simulink model "Harmonic_Restrain_Relay"  (R2024a)
settings: Solver=VariableStepAuto  StartTime=0.0  StopTime=1  EnableMultiTasking=on
libraries: spsFourierLib x4, spsThreePhaseVIMeasurementLib x2, spsThreePhaseBreakerLib x2, spsThreePhaseFaultLib x2, spsCurrentMeasurementLib x1, spsGroundLib x1, spsThreePhaseSeriesRLCBranchLib x1, spsThreePhaseTransformerTwoWindingsLib x1, spsThreePhaseSourceLib x1, spspowerguiLib x1
settings Model: Creator=hp  LastModifiedBy=hp
settings SolverCC: MaxZcPerStep=1
settings DataIOCC: LimitDataPoints=on  MaxDataPoints=10000
settings OptimizationCC: ReuseModelBlockBuffer=off  LifeSpan=inf
settings DebuggingCC: UnconnectedInputMsg=warning  UnconnectedOutputMsg=warning  UnconnectedLineMsg=warning  AllowSymbolicDim=off  SFUnexpectedBacktrackingDiag=warning  SFNoUnconditionalDefaultTransitionDiag=warning  SFExecutionAtInitializationDiag=none  ArithmeticOperatorsInVariantConditions=warning
settings ModelReferenceCC: EnableRefExpFcnMdlSchedulingChecks=on
settings SFSimCC: SimUseLocalCustomCode=off  CustomCodeUndefinedFunction=UseInterfaceOnly
settings RTWCC: RTWUseLocalCustomCode=off  GPUComputeCapability=3.5  DLArmComputeVersion=19.05
settings CodeAppCC: StateflowObjectComments=on
settings GRTTargetCC: TargetLangStandard=C89/C90 (ANSI)
settings ConfigComp: CovMetricSettings=dw  CovSaveCumulativeToWorkspaceVar=on  CovSaveSingleToWorkspaceVar=on  CovExternalEMLEnable=off  CovSFcnEnable=off
settings SimscapeCC: SimscapeLogType=all  SimscapeLogDataHistory=10000

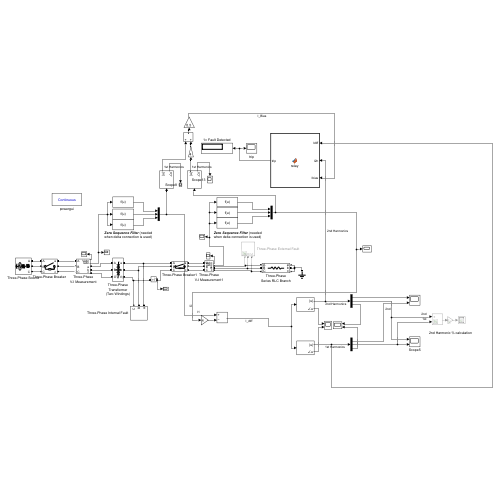
[thumbnail: Simulink's stored preview of the top-level diagram]
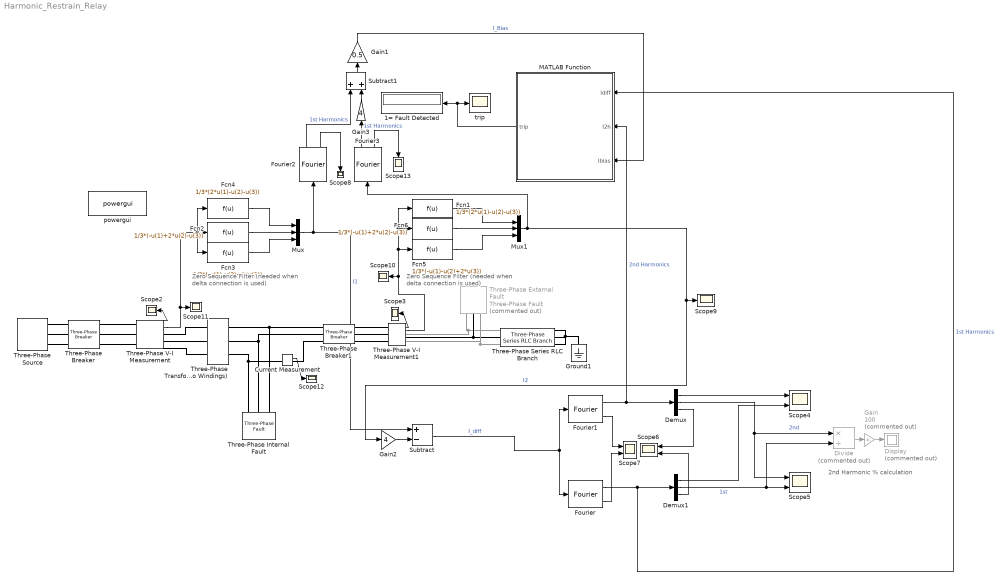
== system Harmonic_Restrain_Relay ==
  note: 2nd Harmonic % calculation
  note: Zero Sequence Filter (needed when delta connection is used)
  note: Zero Sequence Filter (needed when delta connection is used)
  1= Fault Detected : Display
  Current Measurement : spsCurrentMeasurementLib/Current Measurement  PhasorSimulation=off  OutputType=Complex  PSBequivalent=0
  Demux : Demux  Outputs=3
  Demux1 : Demux  Outputs=3
  Display : Display  Commented=on
  Divide : Product  Commented=on  Inputs=*/
  Fcn1 : Fcn  Expr=1/3*(2*u(1)-u(2)-u(3))
  Fcn2 : Fcn  Expr=1/3*(-u(1)+2*u(2)-u(3))
  Fcn3 : Fcn  Expr=1/3*(-u(1)-u(2)+2*u(3))
  Fcn4 : Fcn  Expr=1/3*(2*u(1)-u(2)-u(3))
  Fcn5 : Fcn  Expr=1/3*(-u(1)-u(2)+2*u(3))
  Fcn6 : Fcn  Expr=1/3*(-u(1)+2*u(2)-u(3))
  Fourier : spsFourierLib/Fourier  Freq=60  n=1  InInit=[0, 0]  Ts=0
  Fourier1 : spsFourierLib/Fourier  Freq=60  n=2  InInit=[0, 0]  Ts=0
  Fourier2 : spsFourierLib/Fourier  Freq=60  n=1  InInit=[0, 0]  Ts=0
  Fourier3 : spsFourierLib/Fourier  Freq=60  n=1  InInit=[0, 0]  Ts=0
  Gain : Gain  Commented=on  Gain=100
  Gain1 : Gain  Gain=0.5
  Gain2 : Gain  Gain=4
  Gain3 : Gain  Gain=4
  Ground1 : spsGroundLib/Ground  LConnTagsString=a
  MATLAB Function : MATLAB Function  TreatAsAtomicUnit=on
  Mux : Mux  Inputs=3
  Mux1 : Mux  Inputs=3
  Scope{2..3,8..13} (8 alike) : Scope
  Scope{4..7} (4 alike) : Scope  NumInputPorts=2
  Subtract : Sum  Inputs=+-
  Subtract1 : Sum
  Three-Phase Series RLC Branch : spsThreePhaseSeriesRLCBranchLib/Three-Phase Series RLC Branch  LConnTagsString=A|B|C  RConnTagsString=A|B|C  BranchType=R  Resistance=150  Inductance=0  Capacitance=0  Measurements=None
  Three-Phase Transformer (Two Windings) : spsThreePhaseTransformerTwoWindingsLib/Three-Phase Transformer (Two Windings)  Winding1Connection=Yg  Winding2Connection=Yg  CoreType=Three single-phase transformers  SetSaturation=on  Hysteresis=off  DataFile='hysteresis'  SetInitialFlux=on  Measurements=None  UNITS=pu  NominalPower=[ 150e6 , 60 ]  Winding1=[33000 0.002 0.08]  Winding2=[1.32e+05 0.002 0.08]  Rm=500  Lm=500  L0=25.964  Saturation=[0 0; 0.002 1.2; 0.05 1.35; 0.5 1.45]  InitialFluxes=[0.8 -0.4 -0.4]  BreakLoop=off  DiscreteSolver=Trapezoidal iterative  DataType=off  TransfoNumber=1
  Three-Phase V-I Measurement : spsThreePhaseVIMeasurementLib/Three-Phase V-I Measurement  VoltageMeasurement=phase-to-ground  SetLabelV=off  LabelV=Vabc  Vpu=off  VpuLL=off  CurrentMeasurement=yes  SetLabelI=off  LabelI=Iabc  Ipu=off  Pbase=100e6  Vbase=500e3  OutputType=Complex  PhasorSimulation=off  PSBequivalent=0
  Three-Phase V-I Measurement1 : spsThreePhaseVIMeasurementLib/Three-Phase V-I Measurement  VoltageMeasurement=phase-to-ground  SetLabelV=off  LabelV=Vabc  Vpu=off  VpuLL=off  CurrentMeasurement=yes  SetLabelI=off  LabelI=Iabc  Ipu=off  Pbase=100e6  Vbase=500e3  OutputType=Complex  PhasorSimulation=off  PSBequivalent=0
  Three-Phase Breaker : spsThreePhaseBreakerLib/Three-Phase Breaker  InitialState=open  SwitchA=on  SwitchB=on  SwitchC=on  SwitchTimes=[0, 10]  External=off  BreakerResistance=0.01  SnubberResistance=500  SnubberCapacitance=0.05e-6  Measurements=None
  Three-Phase Breaker1 : spsThreePhaseBreakerLib/Three-Phase Breaker  InitialState=open  SwitchA=on  SwitchB=on  SwitchC=on  SwitchTimes=[0.1 10]  External=off  BreakerResistance=0.01  SnubberResistance=1e6  SnubberCapacitance=inf  Measurements=None
  Three-Phase External Fault : spsThreePhaseFaultLib/Three-Phase Fault  Commented=on  InitialStates=0  FaultA=on  FaultB=on  FaultC=on  GroundFault=on  SwitchTimes=[0.05 10]  External=off  SwitchStatus=NaN  FaultResistance=0.001  GroundResistance=0.01  SnubberResistance=1e6  SnubberCapacitance=inf  Measurements=None
  Three-Phase Internal Fault : spsThreePhaseFaultLib/Three-Phase Fault  InitialStates=0  FaultA=on  FaultB=on  FaultC=on  GroundFault=on  SwitchTimes=[0.4 10]  External=off  SwitchStatus=NaN  FaultResistance=0.001  GroundResistance=0.01  SnubberResistance=1e6  SnubberCapacitance=inf  Measurements=None
  Three-Phase Source : spsThreePhaseSourceLib/Three-Phase Source  InternalConnection=Yg  VoltagePhases=off  Voltage=33e3  PhaseAngle=0  Voltage_phases=[25e3 25e3 25e3]/sqrt(3)  PhaseAngles_phases=[0 -120 +120]  Frequency=60  NonIdealSource=on  SpecifyImpedance=off  Resistance=0.8929  Inductance=16.58e-3  ShortCircuitLevel=100e6  BaseVoltage=25e3  XRratio=7  BusType=swing  Pref=10e3  Qref=0  Prefabc=[10e3, 10e3, 10e3]  Qrefabc=[0, 0, 0]  Qmin=-inf  Qmax=inf
  powergui : spspowerguiLib/powergui  Priority=1  SimulationMode=Continuous  SampleTime=1e-4  frequency=60  Iterations=50  frequencyindice=60  Pbase=100e6  ErrMax=1e-4  UnitsV=kV  UnitsW=MW  buscounter=0  FunctionMessages=off  echomessages=off  EnableUseOfTLC=off  CurrentSourceSwitches=off  DisableSnubberDevices=off  DisableRonSwitches=off  DisableVfSwitches=off  DisplayEquations=off  AutomaticDiscreteSolvers=off  SolverType=Tustin/Backward Euler (TBE)  Interpol=off  ExternalGateDelay=off  methode=off  Ts=100  x0status=blocks  SPID=on  SwTol=0  HookPort=off  NonlinearTolerance=0  nMaxIteration=15  ContinueOnMaxIteration=off  RestoreLinks=warning  ResistiveCurrentMeasurement=off  Frange=[0:2:500]  Ylog=off  Xlog=on  ShowGrid=off  save=off  variable=ZData  structure=0  ZoomFFT=off  StartTime=0.0  cycles=1  DisplayStyle=1  fundamental=60  FreqAxis=off  MaxFrequency=1000  frequencyindicesteady=1  RmsSteady=1  display=off
  trip : Scope
  wires:
  Three-Phase V-I Measurement/2 -> Fcn3/1, Fcn4/1, Fcn2/1, Scope11/1
  Three-Phase V-I Measurement1/2 -> Scope10/1, Fcn5/1, Fcn6/1, Fcn1/1
  Fcn4/1 -> Mux/1
  Fcn2/1 -> Mux/2
  Fcn3/1 -> Mux/3
  Fcn1/1 -> Mux1/1
  Fcn6/1 -> Mux1/2
  Fcn5/1 -> Mux1/3
  Mux1/1 -> Gain2/1, Scope9/1, Fourier3/1  "I2"
  Subtract/1 -> Fourier1/1, Fourier/1  "I_diff"
  Three-Phase V-I Measurement1/1 -> Scope3/1
  Three-Phase V-I Measurement/1 -> Scope2/1
  Fourier/1 -> Demux1/1, MATLAB Function/1(Idiff)  "1st Harmonics"
  Fourier1/1 -> Demux/1, MATLAB Function/2(I2h)  "2nd Harmonics"
  Fourier/2 -> Scope7/2
  Fourier1/2 -> Scope7/1
  Demux1/1 -> Scope4/2
  Demux/1 -> Scope4/1
  Demux/2 -> Divide/1, Scope5/1  "2nd"
  Demux1/3 -> Scope6/2
  Demux1/2 -> Divide/2, Scope5/2  "1st"
  Demux/3 -> Scope6/1
  Current Measurement/1 -> Scope12/1
  Divide/1 -> Gain/1
  Gain/1 -> Display/1
  Fourier2/1 -> Subtract1/1  "1st Harmonics"
  Fourier3/1 -> Gain3/1  "1st Harmonics"
  Subtract1/1 -> Gain1/1
  MATLAB Function/1(trip) -> trip/1, 1= Fault Detected/1
  Mux/1 -> Subtract/1, Fourier2/1  "I1"
  Fourier2/2 -> Scope8/1
  Fourier3/2 -> Scope13/1
  Gain2/1 -> Subtract/2
  Gain3/1 -> Subtract1/2
  Gain1/1 -> MATLAB Function/3(Ibias)  "I_Bias"
  connections:
  Three-Phase Source/RConn1 -- Three-Phase Breaker/LConn1
  Three-Phase Breaker/LConn2 -- Three-Phase Source/RConn2
  Three-Phase Breaker/LConn3 -- Three-Phase Source/RConn3
  Three-Phase Breaker/RConn1 -- Three-Phase V-I Measurement/LConn1
  Three-Phase Breaker/RConn2 -- Three-Phase V-I Measurement/LConn2
  Three-Phase Breaker/RConn3 -- Three-Phase V-I Measurement/LConn3
  Three-Phase V-I Measurement/RConn1 -- Three-Phase Transformer (Two Windings)/LConn1
  Three-Phase V-I Measurement/RConn2 -- Three-Phase Transformer (Two Windings)/LConn2
  Three-Phase V-I Measurement/RConn3 -- Three-Phase Transformer (Two Windings)/LConn3
  Three-Phase Breaker1/LConn1 -- Three-Phase Internal Fault/LConn1 -- Three-Phase Transformer (Two Windings)/RConn1
  Three-Phase Breaker1/LConn2 -- Three-Phase Transformer (Two Windings)/RConn2 -- Three-Phase Internal Fault/LConn2
  Current Measurement/RConn1 -- Three-Phase Breaker1/LConn3
  Three-Phase V-I Measurement1/LConn3 -- Three-Phase Breaker1/RConn3
  Three-Phase V-I Measurement1/LConn2 -- Three-Phase Breaker1/RConn2
  Three-Phase V-I Measurement1/LConn1 -- Three-Phase Breaker1/RConn1
  Three-Phase Series RLC Branch/RConn1 -- Three-Phase Series RLC Branch/RConn3 -- Three-Phase Series RLC Branch/RConn2 -- Ground1/LConn1
  Current Measurement/LConn1 -- Three-Phase Transformer (Two Windings)/RConn3 -- Three-Phase Internal Fault/LConn3
  Three-Phase External Fault/LConn1 -- Three-Phase V-I Measurement1/RConn1 -- Three-Phase Series RLC Branch/LConn1
  Three-Phase Series RLC Branch/LConn2 -- Three-Phase V-I Measurement1/RConn2 -- Three-Phase External Fault/LConn2
  Three-Phase External Fault/LConn3 -- Three-Phase V-I Measurement1/RConn3 -- Three-Phase Series RLC Branch/LConn3

== matlab function Harmonic_Restrain_Relay/MATLAB Function ==
  data: Idiff input; trip output; I2h input; Ibias input
function trip = relay(Idiff, I2h, Ibias)

% Transformer differential protection relay with 2nd Harmonic Restraint
% Inputs: 3-phase current magnitudes in amperes (peak)

% Transformer ratings
S  = 150e6; % 150 MVA
V1 = 33e3;  % 33 kV

% Rated current base (peak amperes)
Ibase = sqrt(2)*S/(sqrt(3)*V1);

% Relay settings
Ipu     = 0.2;     % 20% minimum pickup current
slope   = 0.3;     % 30% percentage differential slope
ratioTh = 0.15;    % 15% second harmonic threshold for inrush restraint
Ihigh   = 8.0;     % 8.0 pu unrestrained instantaneous high-set

% Convert inputs to column vectors and normalize to per-unit
d = abs(Idiff(:))/Ibase;
h = abs(I2h(:))/Ibase;
b = abs(Ibias(:))/Ibase;

% Percentage differential operating condition
pickup  = max(Ipu, slope.*b);
operate = d > pickup;

% Second harmonic restraint with Cross-Phase (Common) Blocking
% When energizing a 3-phase transformer, inrush flux is non-uniform across phases.
% Standard protection practice blocks tripping if 2nd harmonic exceeds ratioTh on any phase.
inrushPhase = (d > 0.5*Ipu) & (h > ratioTh.*d);
inrush = any(inrushPhase);

% High-set instantaneous protection bypasses harmonic restraint
highSet = d > Ihigh;

% Final trip decision
phaseTrip = highSet | (operate & ~inrush);
trip = double(any(phaseTrip));

end
